simulink model "Dynamic_Model"  (R2024b)
settings: Solver=VariableStepAuto  StartTime=0.0  StopTime=10.0  RelTol=1e-3
libraries: matrix_library x2
settings Model: Creator=emrec  LastModifiedBy=emrec

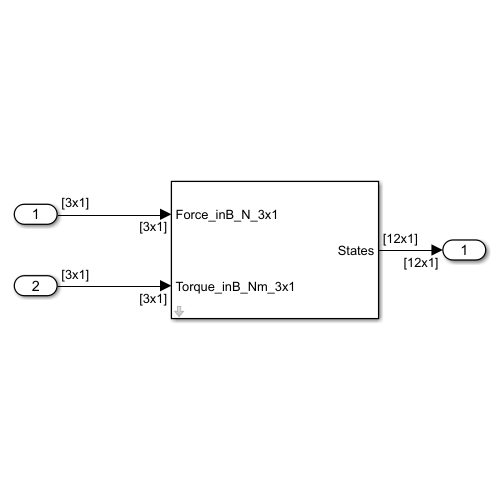
[thumbnail: Simulink's stored preview of the top-level diagram]
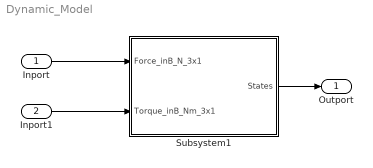
== system Dynamic_Model ==
  Inport : Inport  PortDimensions=[3, 1]
  Inport1 : Inport  Port=2  PortDimensions=[3, 1]
  Subsystem1 : Subsystem  mask{init_states=zeros(12,1), J_B_B=[1 0 0; 0 1 0; 0 0 1], m=1}
      mask prompts: init_states "Initial state values"; J_B_B "Inertia matrix (Kg.m^2)"; m "Mass (Kg)"
  Outport : Outport
  wires:
  Subsystem1/1(States) -> Outport/1
  Inport/1 -> Subsystem1/1(Force_inB_N_3x1)
  Inport1/1 -> Subsystem1/2(Torque_inB_Nm_3x1)

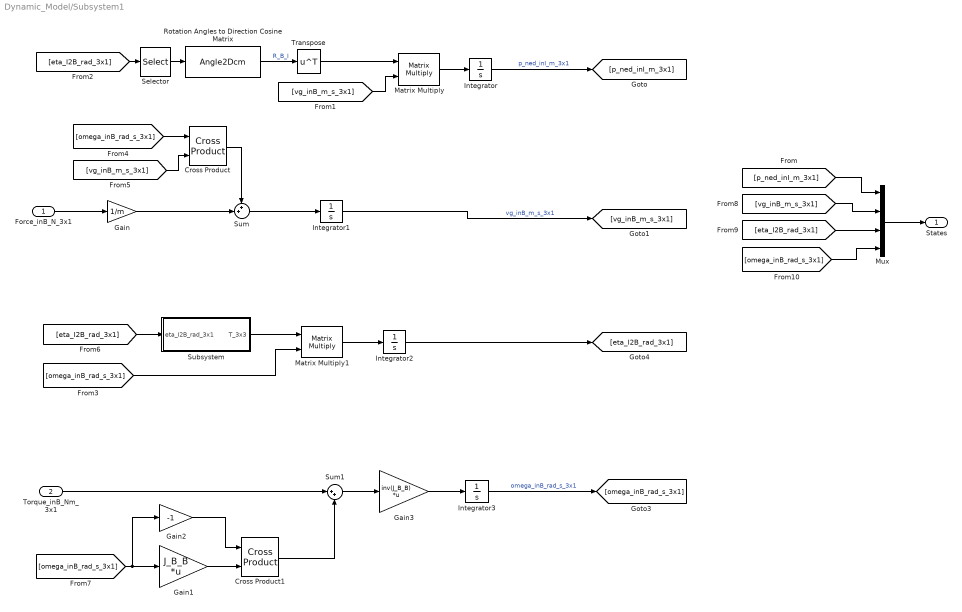
== system Dynamic_Model/Subsystem1 ==
  Force_inB_N_3x1 : Inport
  Torque_inB_Nm_3x1 : Inport  Port=2
  Cross Product : matrix_library/Cross Product
  Cross Product1 : matrix_library/Cross Product
  Gain : Gain  Gain=1/m
  Gain1 : Gain  Gain=J_B_B  Multiplication=Matrix(K*u)
  Gain2 : Gain  Gain=-1
  Gain3 : Gain  Gain=inv(J_B_B)  Multiplication=Matrix(K*u)
  Integrator : Integrator  InitialCondition=init_states(1:3)
  Integrator1 : Integrator  InitialCondition=init_states(4:6)
  Integrator2 : Integrator  InitialCondition=init_states(7:9)
  Integrator3 : Integrator  InitialCondition=init_states(10:12)
  Matrix Multiply : Product  Multiplication=Matrix(*)
  Matrix Multiply1 : Product  Multiplication=Matrix(*)
  Mux : Mux
  Rotation Angles to Direction Cosine Matrix : Angle2Dcm
      settings: AttributesFormatString=Rotation Order: %<rotationOrder>
  Selector : Selector  InputPortWidth=3  IndexOptions=Index vector (dialog)  Indices=[3;2;1]  OutputSizes=1
  Subsystem : Subsystem
  Sum : Sum  Inputs=++|
  Sum1 : Sum  Inputs=|++
  Transpose : Math  Operator=transpose
  States : Outport
  wires:
  Gain3/1 -> Integrator3/1
  [p_ned_inI_m_3x1] -> Mux/1
  [omega_inB_rad_s_3x1] -> Cross Product/1
  Matrix Multiply1/1 -> Integrator2/1
  Gain1/1 -> Cross Product1/2
  [eta_I2B_rad_3x1] -> Subsystem/1(eta_I2B_rad_3x1)
  [omega_inB_rad_s_3x1] -> Matrix Multiply1/2
  Force_inB_N_3x1/1 -> Gain/1
  Integrator1/1 -> [vg_inB_m_s_3x1]  "vg_inB_m_s_3x1"
  [vg_inB_m_s_3x1] -> Cross Product/2
  Selector/1 -> Rotation Angles to Direction Cosine Matrix/1
  [eta_I2B_rad_3x1] -> Selector/1
  Cross Product/1 -> Sum/1
  Integrator/1 -> [p_ned_inI_m_3x1]  "p_ned_inI_m_3x1"
  Matrix Multiply/1 -> Integrator/1
  Gain/1 -> Sum/2
  Rotation Angles to Direction Cosine Matrix/1 -> Transpose/1  "R_B_I"
  [omega_inB_rad_s_3x1] -> Gain2/1, Gain1/1
  Mux/1 -> States/1
  [omega_inB_rad_s_3x1] -> Mux/4
  Transpose/1 -> Matrix Multiply/1
  Integrator3/1 -> [omega_inB_rad_s_3x1]  "omega_inB_rad_s_3x1"
  [vg_inB_m_s_3x1] -> Matrix Multiply/2
  Sum/1 -> Integrator1/1
  [eta_I2B_rad_3x1] -> Mux/3
  Torque_inB_Nm_3x1/1 -> Sum1/1
  Gain2/1 -> Cross Product1/1
  Sum1/1 -> Gain3/1
  Integrator2/1 -> [eta_I2B_rad_3x1]
  [vg_inB_m_s_3x1] -> Mux/2
  Subsystem/1(T_3x3) -> Matrix Multiply1/1
  Cross Product1/1 -> Sum1/2

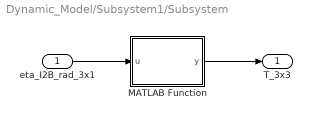
== system Dynamic_Model/Subsystem1/Subsystem ==
  eta_I2B_rad_3x1 : Inport
  MATLAB Function : MATLAB Function  TreatAsAtomicUnit=on
  T_3x3 : Outport
  wires:
  eta_I2B_rad_3x1/1 -> MATLAB Function/1(u)
  MATLAB Function/1(y) -> T_3x3/1

== matlab function Dynamic_Model/Subsystem1/Subsystem/MATLAB Function ==
  data: u input; y output
function y = fcn(u)
    sphi = sin(u(1));
    cphi = cos(u(1));

    sthe = sin(u(2));
    cthe = cos(u(2));

    scthe = 1 / cthe;
    tthe = scthe * sthe;

    y = [1 sphi * tthe cphi*tthe;
         0 cphi -sphi;
         0 sphi*scthe cphi*scthe];
